simulink model "HPP"  (R2026a)
settings: Solver=ode1  StopTime=p.sim.Tstop  FixedStep=HPP_Tnet
model workspace (MAT data in the model file):
  HPP_Tnet = 0.001
  HPP_Ts = 0.001
  HPP_delays = 1
  HPP_f0 = 50
  HPP_network = 1
  HPP_simscape = 1
  buildInfo : object (value not decoded)
undefined symbols (not defined in the file): p
libraries: ee_lib x57, nesl_utility x29, fl_lib x6
(part 5 of 5)

== matlab function HPP/Network/Network model/Simscape/converter 4/current ==
  data: I_re input; Imag output; I_im input; Ib input; Iph output
function [Imag, Iph] = current(I_re, I_im, Ib)
%#codegen
% current phasor (system pu, network angle) -> rms magnitude [A] and phase [rad]
I = complex(I_re, I_im);
Imag = abs(I) * Ib;
Iph = angle(I);
end

== matlab function HPP/Network/Network model/Simscape/converter 4/phasor/space phasor ==
  data: v input; V_re output; t input; Vn input; w0 input; V_im output
function [V_re, V_im] = phasor(v, t, Vn, w0)
%#codegen
% space phasor at the nominal frequency: exact phasor in frequency-and-time mode;
% in time (EMT) mode the instantaneous space phasor (filtered after this block)
a = complex(-0.5, sqrt(3)/2);
s = 2/3*(v(1) + a*v(2) + a^2*v(3)) * exp(complex(0, pi/2 - w0*t));
V = s * sqrt(3/2) / Vn;
V_re = real(V);
V_im = imag(V);
end

== matlab function HPP/Network/Network model/Simscape/converter 5/current ==
  data: I_re input; Imag output; I_im input; Ib input; Iph output
function [Imag, Iph] = current(I_re, I_im, Ib)
%#codegen
% current phasor (system pu, network angle) -> rms magnitude [A] and phase [rad]
I = complex(I_re, I_im);
Imag = abs(I) * Ib;
Iph = angle(I);
end

== matlab function HPP/Network/Network model/Simscape/converter 5/phasor/space phasor ==
  data: v input; V_re output; t input; Vn input; w0 input; V_im output
function [V_re, V_im] = phasor(v, t, Vn, w0)
%#codegen
% space phasor at the nominal frequency: exact phasor in frequency-and-time mode;
% in time (EMT) mode the instantaneous space phasor (filtered after this block)
a = complex(-0.5, sqrt(3)/2);
s = 2/3*(v(1) + a*v(2) + a^2*v(3)) * exp(complex(0, pi/2 - w0*t));
V = s * sqrt(3/2) / Vn;
V_re = real(V);
V_im = imag(V);
end

== matlab function HPP/Network/Network model/Simscape/HPP bus voltage/phasor/space phasor ==
  data: v input; V_re output; t input; Vn input; w0 input; V_im output
function [V_re, V_im] = phasor(v, t, Vn, w0)
%#codegen
% space phasor at the nominal frequency: exact phasor in frequency-and-time mode;
% in time (EMT) mode the instantaneous space phasor (filtered after this block)
a = complex(-0.5, sqrt(3)/2);
s = 2/3*(v(1) + a*v(2) + a^2*v(3)) * exp(complex(0, pi/2 - w0*t));
V = s * sqrt(3/2) / Vn;
V_re = real(V);
V_im = imag(V);
end

== matlab function HPP/Network/Network model/Simscape/POC voltage/phasor/space phasor ==
  data: v input; V_re output; t input; Vn input; w0 input; V_im output
function [V_re, V_im] = phasor(v, t, Vn, w0)
%#codegen
% space phasor at the nominal frequency: exact phasor in frequency-and-time mode;
% in time (EMT) mode the instantaneous space phasor (filtered after this block)
a = complex(-0.5, sqrt(3)/2);
s = 2/3*(v(1) + a*v(2) + a^2*v(3)) * exp(complex(0, pi/2 - w0*t));
V = s * sqrt(3/2) / Vn;
V_re = real(V);
V_im = imag(V);
end

== matlab function HPP/Network/Network model/Simscape/converter 1/current ==
  data: I_re input; Imag output; I_im input; Ib input; Iph output
function [Imag, Iph] = current(I_re, I_im, Ib)
%#codegen
% current phasor (system pu, network angle) -> rms magnitude [A] and phase [rad]
I = complex(I_re, I_im);
Imag = abs(I) * Ib;
Iph = angle(I);
end

== matlab function HPP/Network/Network model/Nodal/solve ==
  data: I_re input; V_re output; I_im input; E input; Zre input; Zim input; Zg_ri input; brZre input; brZim input; brB input; theta input; V_im output; P_plant output; Q_plant output; V_bus output; P_poc output; Q_poc output; V_poc output; V_bus_re output; V_bus_im output; V_poc_re output; V_poc_im output; net parameter
function [V_re, V_im, P_plant, Q_plant, V_bus, P_poc, Q_poc, V_poc, V_bus_re, V_bus_im, V_poc_re, V_poc_im] = solve(I_re, I_im, E, Zre, Zim, Zg_ri, brZre, brZim, brB, theta, net)
%#codegen
% numeric network data come in as (tunable) inputs; net holds the structure
Z  = complex(Zre, Zim);
nA = numel(I_re);
n  = size(Z, 1);
Zg = complex(Zg_ri(1), Zg_ri(2));
I = complex(zeros(n, 1), zeros(n, 1));
I(1:nA) = complex(I_re(:), I_im(:));
Ec = E * exp(1i * theta);                 % grid source, rotated by the grid angle (Grid frequency)
I(net.poc) = I(net.poc) + Ec / Zg;        % grid Norton source at the POC (E: grid voltage, incl. dips)
V = Z * I;
V_re = real(V(1:nA));
V_im = imag(V(1:nA));
% power each plant delivers into the HPP busbar (its measurement point):
% flows of its plant branches at the busbar end, incl. bus-end charging
Vb = V(net.bus);
Ibr = (V(net.brFrom) - Vb) ./ complex(brZre, brZim) - 1i * brB .* Vb;
Sbr = Vb .* conj(Ibr);
P_plant = zeros(3, 1);  Q_plant = zeros(3, 1);
for j = 1:numel(Sbr)
    P_plant(net.brPlant(j)) = P_plant(net.brPlant(j)) + real(Sbr(j));
    Q_plant(net.brPlant(j)) = Q_plant(net.brPlant(j)) + imag(Sbr(j));
end
V_bus = abs(Vb);
Vp = V(net.poc);
Spoc = Vp * conj((Vp - Ec) / Zg);         % power into the grid
P_poc = real(Spoc);  Q_poc = imag(Spoc);  V_poc = abs(Vp);
% busbar and POC voltage phasors for the frequency measurement (PLLs)
V_bus_re = real(Vb);  V_bus_im = imag(Vb);
V_poc_re = real(Vp);  V_poc_im = imag(Vp);
end

== matlab function HPP/Network/Network model/Simscape/converter 1/phasor/space phasor ==
  data: v input; V_re output; t input; Vn input; w0 input; V_im output
function [V_re, V_im] = phasor(v, t, Vn, w0)
%#codegen
% space phasor at the nominal frequency: exact phasor in frequency-and-time mode;
% in time (EMT) mode the instantaneous space phasor (filtered after this block)
a = complex(-0.5, sqrt(3)/2);
s = 2/3*(v(1) + a*v(2) + a^2*v(3)) * exp(complex(0, pi/2 - w0*t));
V = s * sqrt(3/2) / Vn;
V_re = real(V);
V_im = imag(V);
end

== matlab function HPP/Network/Network model/Simscape/converter 2/current ==
  data: I_re input; Imag output; I_im input; Ib input; Iph output
function [Imag, Iph] = current(I_re, I_im, Ib)
%#codegen
% current phasor (system pu, network angle) -> rms magnitude [A] and phase [rad]
I = complex(I_re, I_im);
Imag = abs(I) * Ib;
Iph = angle(I);
end

== matlab function HPP/Network/Network model/Simscape/converter 2/phasor/space phasor ==
  data: v input; V_re output; t input; Vn input; w0 input; V_im output
function [V_re, V_im] = phasor(v, t, Vn, w0)
%#codegen
% space phasor at the nominal frequency: exact phasor in frequency-and-time mode;
% in time (EMT) mode the instantaneous space phasor (filtered after this block)
a = complex(-0.5, sqrt(3)/2);
s = 2/3*(v(1) + a*v(2) + a^2*v(3)) * exp(complex(0, pi/2 - w0*t));
V = s * sqrt(3/2) / Vn;
V_re = real(V);
V_im = imag(V);
end

== matlab function HPP/Network/Network model/Simscape/converter 3/current ==
  data: I_re input; Imag output; I_im input; Ib input; Iph output
function [Imag, Iph] = current(I_re, I_im, Ib)
%#codegen
% current phasor (system pu, network angle) -> rms magnitude [A] and phase [rad]
I = complex(I_re, I_im);
Imag = abs(I) * Ib;
Iph = angle(I);
end
